simulink model "fir_tap_test"  (Simulink 7.2)
settings: Solver=VariableStepDiscrete  StartTime=0.0  StopTime=1000  RelTol=1e-3
libraries: xbsIndex_r4 x9, casper_library_downconverter x1
settings Model: Creator=User  LastModifiedBy=root
settings OptimizationCC: InitFltsAndDblsToZero=on
settings DebuggingCC: SaveWithDisabledLinksMsg=none  SaveWithParameterizedLinksMsg=none

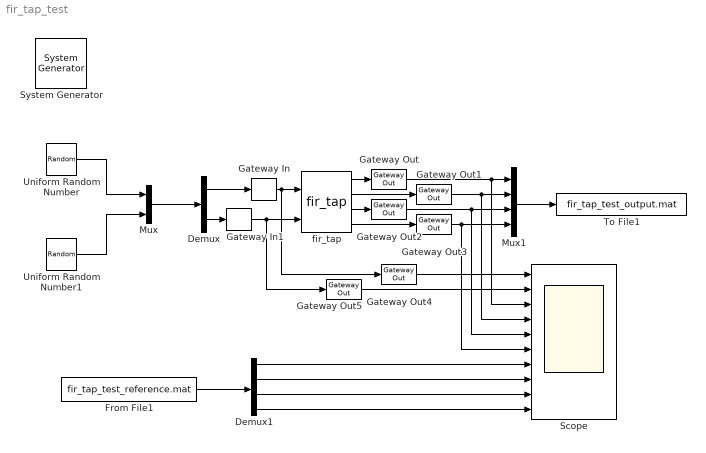
== system fir_tap_test ==
  " System Generator" : xbsIndex_r4/ System Generator  Tag=genX  SystemSampleTime=-1  xilinxfamily=Virtex4  part=xc4vsx35  speed=-10  package=ff668  synthesis_tool=XST  clock_wrapper=Clock Enables  directory=./netlist  testbench=off  simulink_period=1  sysclk_period=100  dcm_input_clock_period=100  incr_netlist=off  trim_vbits=Everywhere in SubSystem  dbl_ovrd=According to Block Masks  core_generation=According to Block Masks  run_coregen=off  deprecated_control=off  eval_field=0  block_type=sysgen
      settings: block_version=10.1.1
  Demux : Demux  Outputs=2
  Demux1 : Demux
  From File1 : FromFile  FileName=fir_tap_test_reference.mat  SampleTime=1
  Gateway In : xbsIndex_r4/Gateway In  arith_type="Signed  (2's comp)"  n_bits=16  bin_pt=14  quantization=Truncate  overflow=Wrap  period=1  dbl_ovrd=off  timing_constraint=None  locs_specified=off  LOCs={}  hdl_port=on  block_type=gatewayin
      settings: infoedit="Gateway in block.  Converts inputs of type Simulink integer, double and fixed point to  Xilinx fixed point type.<P><P>Hardware notes:  In hardware these blocks become top level input ports."  block_version=10.1.1
  Gateway In1 : xbsIndex_r4/Gateway In  arith_type="Signed  (2's comp)"  n_bits=16  bin_pt=14  quantization=Truncate  overflow=Wrap  period=1  dbl_ovrd=off  timing_constraint=None  locs_specified=off  LOCs={}  hdl_port=on  block_type=gatewayin
      settings: infoedit="Gateway in block.  Converts inputs of type Simulink integer, double and fixed point to  Xilinx fixed point type.<P><P>Hardware notes:  In hardware these blocks become top level input ports."  block_version=10.1.1
  Gateway Out{,1..5} (6 alike) : xbsIndex_r4/Gateway Out  hdl_port=on  timing_constraint=None  locs_specified=off  LOCs={}  block_type=gatewayout
      settings: infoedit="Gateway out block.  Converts Xilinx fixed point inputs into ouputs of type Simulink integer, double, or fixed point.<P><P>Hardware notes:  In hardware these blocks become top level output ports or are discarded, depending on how they are configured."  block_version=10.1.1
  Mux : Mux  Inputs=2
  Mux1 : Mux
  Scope : Scope  NumInputPorts=10
      settings: YMin=-5~-5~-5~-5~-5~-5~-5~-5~-5~-5  YMax=5~5~5~5~5~5~5~5~5~5
  To File1 : ToFile  Filename=fir_tap_test_output.mat  MatrixName=output
  Uniform Random Number : UniformRandomNumber  SampleTime=0
  Uniform Random Number1 : UniformRandomNumber  Seed=10  SampleTime=0
  fir_tap : casper_library_downconverter/fir_tap  SystemSampleTime=-1  factor=0.12345  latency=2  coeff_bit_width=25  coeff_bin_pt=24
  wires:
  Uniform Random Number/1 -> Mux/1
  Uniform Random Number1/1 -> Mux/2
  Demux/1 -> Gateway In/1
  Demux/2 -> Gateway In1/1
  fir_tap/1 -> Gateway Out/1
  fir_tap/2 -> Gateway Out1/1
  fir_tap/3 -> Gateway Out2/1
  fir_tap/4 -> Gateway Out3/1
  Mux1/1 -> To File1/1
  Gateway In/1 -> fir_tap/1, Gateway Out4/1
  Gateway In1/1 -> fir_tap/2, Gateway Out5/1
  Gateway Out/1 -> Mux1/1, Scope/3
  Gateway Out1/1 -> Mux1/2, Scope/4
  Gateway Out2/1 -> Mux1/3, Scope/5
  Gateway Out3/1 -> Mux1/4, Scope/6
  From File1/1 -> Demux1/1
  Gateway Out4/1 -> Scope/1
  Gateway Out5/1 -> Scope/2
  Demux1/1 -> Scope/7
  Demux1/2 -> Scope/8
  Demux1/3 -> Scope/9
  Demux1/4 -> Scope/10
  Mux/1 -> Demux/1
